simulink model "closed_loop_control"  (R2026b)
settings: Solver=ode45  StopTime=10
settings Model: Creator=Mahdad  LastModifiedBy=Mahdad

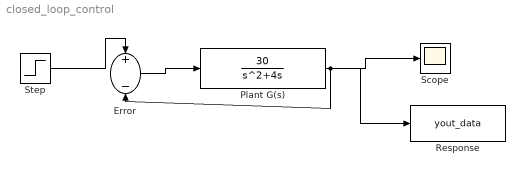
== system closed_loop_control ==
  Error : Sum  Inputs=+-
  Plant G(s) : TransferFcn  Numerator=[30]  Denominator=[1 4 0]
  Response : ToWorkspace  VariableName=yout_data  SaveFormat=Timeseries  SampleTime=-1
  Scope : Scope
  Step : Step  Time=0  SampleTime=0
  wires:
  Step/1 -> Error/1
  Error/1 -> Plant G(s)/1
  Plant G(s)/1 -> Scope/1, Response/1, Error/2
